simulink model "H04_ERR"  (R2026a)
settings: Solver=VariableStepAuto  MaxStep=tau/25
InitFcn:
  | K = 5;
  | tau = 0.5;
  | 
  | y_0 = 2.5;
settings Model: Creator=Szalay  LastModifiedBy=Szalay

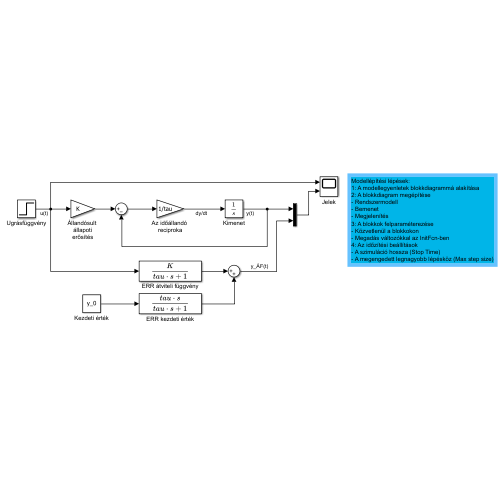
[thumbnail: Simulink's stored preview of the top-level diagram]
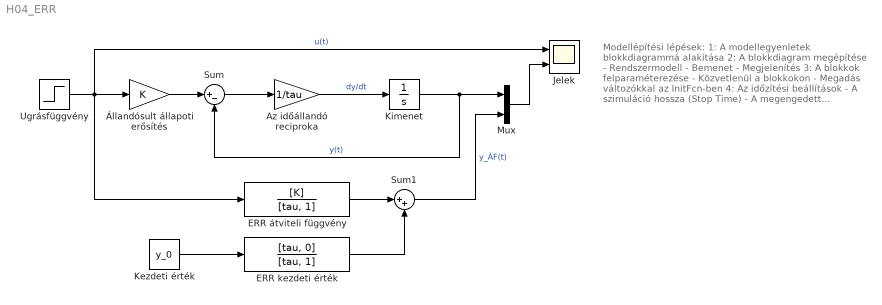
== system H04_ERR ==
  note: Modellépítési lépések:
      | 1: A modellegyenletek blokkdiagrammá alakítása
      | 2: A blokkdiagram megépítése
      | - Rendszermodell
      | - Bemenet
      | - Megjelenítés
      | 3: A blokkok felparaméterezése
      | - Közvetlenül a blokkokon
      | - Megadás változókkal az InitFcn-ben
      | 4: Az időzítési beállítások
      | - A szimuláció hossza (Stop Time)
      | - A megengedett legnagyobb lépésköz (Max step size)
  Az időállandó reciproka : Gain  Gain=1/tau
  ERR kezdeti érték : TransferFcn  Numerator=[tau, 0]  Denominator=[tau, 1]
  ERR átviteli függvény : TransferFcn  Numerator=[K]  Denominator=[tau, 1]
  Jelek : Scope  NumInputPorts=2
      settings: ActiveDisplayYMinimum=-0.62499999999999911  ActiveDisplayYMaximum=5.6249999999999929
  Kezdeti érték : Constant  Value=y_0
  Kimenet : Integrator  InitialCondition=y_0
  Mux : Mux  Inputs=2
  Sum : Sum  Inputs=|+-
  Sum1 : Sum  Inputs=|++
  Ugrásfüggvény : Step  Time=5  SampleTime=0
  Állandósult állapoti erősítés : Gain  Gain=K
  wires:
  Kimenet/1 -> Mux/1, Sum/2  "y(t)"
  Az időállandó reciproka/1 -> Kimenet/1  "dy/dt"
  Sum/1 -> Az időállandó reciproka/1
  Állandósult állapoti erősítés/1 -> Sum/1
  Ugrásfüggvény/1 -> ERR átviteli függvény/1, Jelek/1, Állandósult állapoti erősítés/1  "u(t)"
  Sum1/1 -> Mux/2  "y_ÁF(t)"
  Mux/1 -> Jelek/2
  Kezdeti érték/1 -> ERR kezdeti érték/1
  ERR átviteli függvény/1 -> Sum1/1
  ERR kezdeti érték/1 -> Sum1/2
